simulink model "DABThermalAnalysisWithCustomMOSFET"  (R2026a)
settings: Solver=ode23t  StopTime=0.06  MaxStep=1e-5  AbsTol=1e-3
PreLoadFcn:
  | DABThermalAnalysisWithCustomMOSFETInputParameters;
model workspace (MAT data in the model file):
  ConverterKey : string (value not decoded)
undefined symbols (not defined in the file): DAB, DABController, DABDesign, DiscIntNeverNeededParam, M1p, M1s, M2p, M2s, M3p, M3s, M4p, M4s
libraries: ee_lib x21, nesl_utility x16, fl_lib x11, slpidlib x4, simulink_extras x1
(part 2 of 2)

== system DABThermalAnalysisWithCustomMOSFET/DAB Controller/CC-CV Control/CV Mode/Voltage PI/PIContinuous ==
  error : Inport
  PI Controller : slpidlib/PID Controller  Controller=PI  Form=Parallel  TimeDomain=Continuous-time  UseExternalTs=off  SampleTime=-1  IntegratorMethod=Forward Euler  FilterMethod=Forward Euler  ControllerParametersSource=internal  P=Kpv  I=Kiv  UseKiTs=off  D=0.01  UseExternalDerivativeSource=off  N=100  UseFilter=on  TunerSelectOption=Transfer Function Based (PID Tuner App)  InitialConditionSource=internal  InitialConditionForIntegrator=0  InitialConditionForFilter=0  DifferentiatorICPrevScaledInput=0  ExternalReset=none  TrackingMode=off  Kt=1  LimitOutput=on  SatLimitsSource=internal  UpperSaturationLimit=phaseShiftMax*0.98  LowerSaturationLimit=phaseShiftMin*0.98  LinearizeAsGain=on  AntiWindupMode=clamping  Kb=1  LimitIntegrator=on  UpperIntegratorSaturationLimit=phaseShiftMax*0.98  LowerIntegratorSaturationLimit=phaseShiftMin*0.98  POutMin=[]  POutMax=[]  IOutMin=[]  IOutMax=[]  DOutMin=[]  DOutMax=[]  NOutMin=[]  NOutMax=[]  SumOutMin=[]  SumOutMax=[]  SaturationOutMin=[]  SaturationOutMax=[]  PParamMin=[]  PParamMax=[]  IParamMin=[]  IParamMax=[]  DParamMin=[]  DParamMax=[]  NParamMin=[]  NParamMax=[]  KbParamMin=[]  KbParamMax=[]  KtParamMin=[]  KtParamMax=[]  KbOutMin=[]  KbOutMax=[]  KtOutMin=[]  KtOutMax=[]  IntegratorOutMin=[]  IntegratorOutMax=[]  FilterOutMin=[]  FilterOutMax=[]  SumI1OutMin=[]  SumI1OutMax=[]  SumI2OutMin=[]  SumI2OutMax=[]  SumI3OutMin=[]  SumI3OutMax=[]  SumI4OutMin=[]  SumI4OutMax=[]  SumDOutMin=[]  SumDOutMax=[]  DifferentiatorOutMin=[]  DifferentiatorOutMax=[]  FilterDiffOutCoefMin=[]  FilterDiffOutCoefMax=[]  ReciprocalOutMin=[]  ReciprocalOutMax=[]  SumDenOutMin=[]  SumDenOutMax=[]  SumNumOutMin=[]  SumNumOutMax=[]  DivideOutMin=[]  DivideOutMax=[]  UdiffTsProdOutMin=[]  UdiffTsProdOutMax=[]  NTsProdOutMin=[]  NTsProdOutMax=[]  UintegralTsProdOutMin=[]  UintegralTsProdOutMax=[]  UngainTsProdOutMin=[]  UngainTsProdOutMax=[]  ClampingZeroOutDataTypeStr=Inherit: Inherit via back propagation  ClampingZeroOutMin=[]  ClampingZeroOutMax=[]  FilterDenConstantOutDataTypeStr=Inherit: Inherit via back propagation  FilterDenConstantOutMin=[]  FilterDenConstantOutMax=[]  PCopyOutDataTypeStr=Inherit: Inherit via back propagation  PCopyOutMin=[]  PCopyOutMax=[]  NCopyOutDataTypeStr=Inherit: Inherit via back propagation  NCopyOutMin=[]  NCopyOutMax=[]  IntegratorContinuousStateAttributes=''  IntegratorStateMustResolveToSignalObject=off  IntegratorRTWStateStorageClass=Auto  FilterContinuousStateAttributes=''  FilterStateMustResolveToSignalObject=off  FilterRTWStateStorageClass=Auto  ParallelPVariant=InternalParameters  IdealPVariant=Disabled  IVariant=InternalParameters  DVariant=Disabled  IntegratorVariant=Continuous  SatVariant=Enabled  AWVariant=ContClampingParallel  PCopyVariant=Disabled  TRVariant=Disabled  FdbkBlocksVariant=Forward  IdealPFdbkVariant=Disabled  SatFdbkVariant=Disabled  DerivativeFilterVariant=Disabled  NVariant=Disabled  NCopyVariant=Disabled_SignalSpec  FilterICVariant=Disabled  IntegratorICVariant=InternalICs  ExternalResetVariant=Disabled  TRSumVariant=Passthrough  SumFdbkVariant=Disabled  SumVariant=Sum_PI  TsampFilterVariant=InternalTs  TsampNgainVariant=Passthrough  TsampIntegralVariant=Disabled_SignalSpec  ExternalSaturationOutDataTypeStr=Inherit: Same as second input  DerivativeSourceVariant=Disabled  PreIntVariant=InternalPreInt
  vc : Outport
  wires:
  PI Controller/1 -> vc/1
  error/1 -> PI Controller/1

== system DABThermalAnalysisWithCustomMOSFET/DAB Controller/CC-CV Control/CV Mode/Voltage PI/PIDiscrete ==
  error : Inport
  PI Controller : slpidlib/PID Controller  Controller=PI  Form=Parallel  TimeDomain=Discrete-time  UseExternalTs=off  SampleTime=Ts  IntegratorMethod=Forward Euler  FilterMethod=Forward Euler  ControllerParametersSource=internal  P=Kpv  I=Kiv  UseKiTs=off  D=0  UseExternalDerivativeSource=off  N=100  UseFilter=on  TunerSelectOption=Transfer Function Based (PID Tuner App)  InitialConditionSource=internal  InitialConditionForIntegrator=0  InitialConditionForFilter=0  DifferentiatorICPrevScaledInput=0  ExternalReset=none  TrackingMode=off  Kt=1  LimitOutput=on  SatLimitsSource=internal  UpperSaturationLimit=phaseShiftMax  LowerSaturationLimit=phaseShiftMin  LinearizeAsGain=on  AntiWindupMode=clamping  Kb=1  LimitIntegrator=on  UpperIntegratorSaturationLimit=phaseShiftMax  LowerIntegratorSaturationLimit=phaseShiftMin  POutMin=[]  POutMax=[]  IOutMin=[]  IOutMax=[]  DOutMin=[]  DOutMax=[]  NOutMin=[]  NOutMax=[]  SumOutMin=[]  SumOutMax=[]  SaturationOutMin=[]  SaturationOutMax=[]  PParamMin=[]  PParamMax=[]  IParamMin=[]  IParamMax=[]  DParamMin=[]  DParamMax=[]  NParamMin=[]  NParamMax=[]  KbParamMin=[]  KbParamMax=[]  KtParamMin=[]  KtParamMax=[]  KbOutMin=[]  KbOutMax=[]  KtOutMin=[]  KtOutMax=[]  IntegratorOutMin=[]  IntegratorOutMax=[]  FilterOutMin=[]  FilterOutMax=[]  SumI1OutMin=[]  SumI1OutMax=[]  SumI2OutMin=[]  SumI2OutMax=[]  SumI3OutMin=[]  SumI3OutMax=[]  SumI4OutMin=[]  SumI4OutMax=[]  SumDOutMin=[]  SumDOutMax=[]  DifferentiatorOutMin=[]  DifferentiatorOutMax=[]  FilterDiffOutCoefMin=[]  FilterDiffOutCoefMax=[]  ReciprocalOutMin=[]  ReciprocalOutMax=[]  SumDenOutMin=[]  SumDenOutMax=[]  SumNumOutMin=[]  SumNumOutMax=[]  DivideOutMin=[]  DivideOutMax=[]  UdiffTsProdOutMin=[]  UdiffTsProdOutMax=[]  NTsProdOutMin=[]  NTsProdOutMax=[]  UintegralTsProdOutMin=[]  UintegralTsProdOutMax=[]  UngainTsProdOutMin=[]  UngainTsProdOutMax=[]  ClampingZeroOutDataTypeStr=Inherit: Inherit via back propagation  ClampingZeroOutMin=[]  ClampingZeroOutMax=[]  FilterDenConstantOutDataTypeStr=Inherit: Inherit via back propagation  FilterDenConstantOutMin=[]  FilterDenConstantOutMax=[]  PCopyOutDataTypeStr=Inherit: Inherit via back propagation  PCopyOutMin=[]  PCopyOutMax=[]  NCopyOutDataTypeStr=Inherit: Inherit via back propagation  NCopyOutMin=[]  NCopyOutMax=[]  IntegratorContinuousStateAttributes=''  IntegratorStateMustResolveToSignalObject=off  IntegratorRTWStateStorageClass=Auto  FilterContinuousStateAttributes=''  FilterStateMustResolveToSignalObject=off  FilterRTWStateStorageClass=Auto  ParallelPVariant=InternalParameters  IdealPVariant=Disabled  IVariant=InternalParameters  DVariant=Disabled  IntegratorVariant=Discrete  SatVariant=Enabled  AWVariant=DiscClampingParallel  PCopyVariant=Disabled  TRVariant=Disabled  FdbkBlocksVariant=Forward  IdealPFdbkVariant=Disabled  SatFdbkVariant=Disabled  DerivativeFilterVariant=Disabled  NVariant=Disabled  NCopyVariant=Disabled_SignalSpec  FilterICVariant=Disabled  IntegratorICVariant=InternalICs  ExternalResetVariant=Disabled  TRSumVariant=Passthrough  SumFdbkVariant=Disabled  SumVariant=Sum_PI  TsampFilterVariant=InternalTs  TsampNgainVariant=Passthrough  TsampIntegralVariant=Disabled_SignalSpec  ExternalSaturationOutDataTypeStr=Inherit: Same as second input  DerivativeSourceVariant=Disabled  PreIntVariant=InternalPreInt
  vc : Outport
  wires:
  PI Controller/1 -> vc/1
  error/1 -> PI Controller/1

== system DABThermalAnalysisWithCustomMOSFET/DAB Controller/Output Mode/PWMSignal/Gate Signal Generator/Phase-Shifted Sawtooth ==
  S : Inport
  tPhase : Inport  Port=2
  Ts : Inport  Port=3
  Add : Sum
  Mod : Math  Operator=mod
  PS : Outport
  wires:
  tPhase/1 -> Add/2
  Mod/1 -> PS/1
  Ts/1 -> Mod/2
  Add/1 -> Mod/1
  S/1 -> Add/1

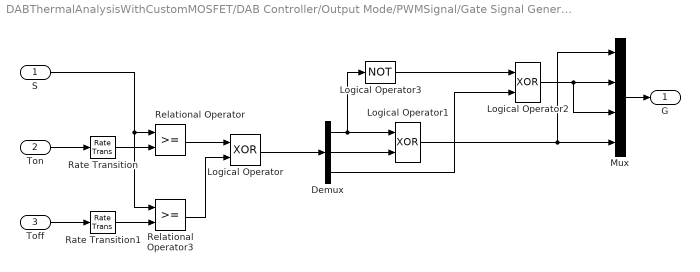
== system DABThermalAnalysisWithCustomMOSFET/DAB Controller/Output Mode/PWMSignal/Gate Signal Generator/Primary Bridge Gate ==
  S : Inport
  Ton : Inport  Port=2
  Toff : Inport  Port=3
  Demux : Demux  Outputs=3
  Logical Operator : Logic  Operator=XOR  AllPortsSameDT=off  OutDataTypeStr=boolean
  Logical Operator1 : Logic  Operator=XOR  AllPortsSameDT=off  OutDataTypeStr=boolean
  Logical Operator2 : Logic  Operator=XOR  AllPortsSameDT=off  OutDataTypeStr=boolean
  Logical Operator3 : Logic  Operator=NOT  AllPortsSameDT=off  OutDataTypeStr=boolean
  Mux : Mux
  Rate Transition : RateTransition
  Rate Transition1 : RateTransition
  Relational Operator : RelationalOperator  OutDataTypeStr=boolean  InputSameDT=off
  Relational Operator3 : RelationalOperator  OutDataTypeStr=boolean  InputSameDT=off
  G : Outport
  wires:
  Mux/1 -> G/1
  Logical Operator1/1 -> Mux/1, Mux/4
  Logical Operator3/1 -> Logical Operator2/1
  Demux/3 -> Logical Operator2/2
  Demux/2 -> Logical Operator1/2
  Demux/1 -> Logical Operator3/1, Logical Operator1/1
  Logical Operator/1 -> Demux/1
  Ton/1 -> Rate Transition/1
  Toff/1 -> Rate Transition1/1
  Rate Transition/1 -> Relational Operator/2
  Relational Operator3/1 -> Logical Operator/2
  Rate Transition1/1 -> Relational Operator3/2
  S/1 -> Relational Operator/1, Relational Operator3/1
  Relational Operator/1 -> Logical Operator/1
  Logical Operator2/1 -> Mux/3, Mux/2

== system DABThermalAnalysisWithCustomMOSFET/DAB Controller/Output Mode/PWMSignal/Gate Signal Generator/Sawtooth Time Generator ==
  Ts : Inport
  Add3 : Sum  Inputs=-+
  Constant2 : Constant
  Discrete-Time Integrator1 : DiscreteIntegrator  ExternalReset=rising  InitialConditionSource=external  SampleTime=-1  ShowStatePort=on  ICPrevOutput=DiscIntNeverNeededParam  ICPrevScaledInput=DiscIntNeverNeededParam
  Initial : InitialCondition  Value=0
  Relational Operator1 : RelationalOperator  Operator=>  OutDataTypeStr=boolean  InputSameDT=off
  TimeRamp : Outport
  wires:
  Initial/1 -> Discrete-Time Integrator1/3
  Add3/1 -> Initial/1
  Discrete-Time Integrator1/State -> Relational Operator1/1, Add3/2
  Ts/1 -> Relational Operator1/2, Add3/1
  Discrete-Time Integrator1/1 -> TimeRamp/1
  Constant2/1 -> Discrete-Time Integrator1/1
  Relational Operator1/1 -> Discrete-Time Integrator1/2

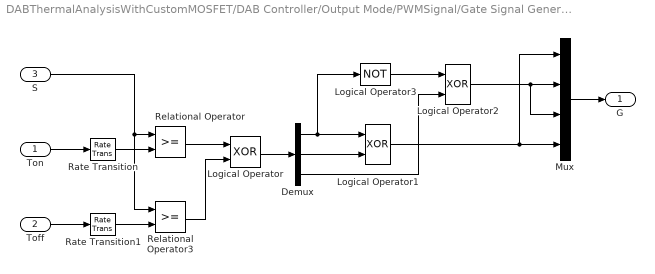
== system DABThermalAnalysisWithCustomMOSFET/DAB Controller/Output Mode/PWMSignal/Gate Signal Generator/Secondary Bridge Gate ==
  Ton : Inport
  Toff : Inport  Port=2
  S : Inport  Port=3
  Demux : Demux  Outputs=3
  Logical Operator : Logic  Operator=XOR  AllPortsSameDT=off  OutDataTypeStr=boolean
  Logical Operator1 : Logic  Operator=XOR  AllPortsSameDT=off  OutDataTypeStr=boolean
  Logical Operator2 : Logic  Operator=XOR  AllPortsSameDT=off  OutDataTypeStr=boolean
  Logical Operator3 : Logic  Operator=NOT  AllPortsSameDT=off  OutDataTypeStr=boolean
  Mux : Mux
  Rate Transition : RateTransition
  Rate Transition1 : RateTransition
  Relational Operator : RelationalOperator  OutDataTypeStr=boolean  InputSameDT=off
  Relational Operator3 : RelationalOperator  OutDataTypeStr=boolean  InputSameDT=off
  G : Outport
  wires:
  Mux/1 -> G/1
  Logical Operator1/1 -> Mux/4, Mux/1
  Logical Operator3/1 -> Logical Operator2/1
  Demux/3 -> Logical Operator2/2
  Demux/2 -> Logical Operator1/2
  Demux/1 -> Logical Operator3/1, Logical Operator1/1
  Logical Operator/1 -> Demux/1
  Ton/1 -> Rate Transition/1
  Toff/1 -> Rate Transition1/1
  Rate Transition/1 -> Relational Operator/2
  Relational Operator3/1 -> Logical Operator/2
  Rate Transition1/1 -> Relational Operator3/2
  S/1 -> Relational Operator/1, Relational Operator3/1
  Relational Operator/1 -> Logical Operator/1
  Logical Operator2/1 -> Mux/2, Mux/3
